simulink model "Shepherd_Battery_Model"  (R2025b)
settings: Solver=ode23  StartTime=0.0  StopTime=1000  MaxStep=0.01  RelTol=1e-4  AbsTol=1e-6
libraries: fl_lib x5, nesl_utility x5
settings Model: Creator=psvan  LastModifiedBy=psvan

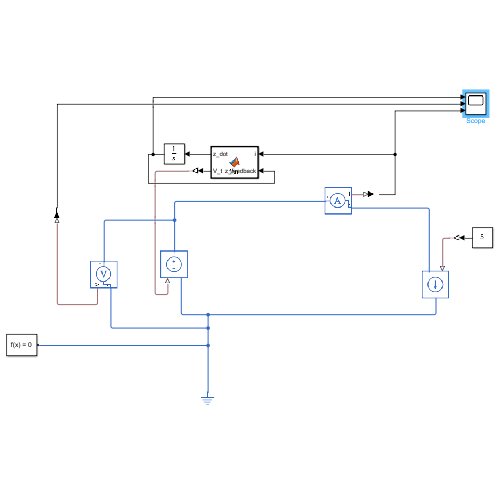
[thumbnail: Simulink's stored preview of the top-level diagram]
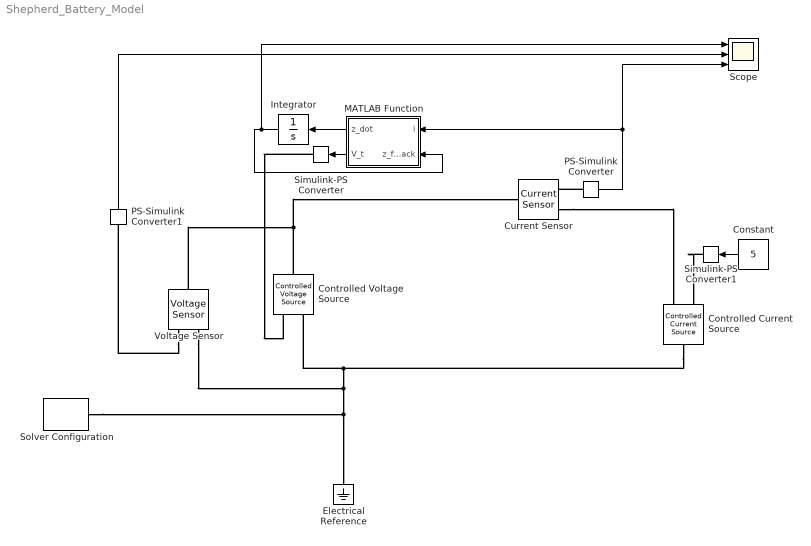
== system Shepherd_Battery_Model ==
  Constant : Constant  Value=5
  Controlled Current Source : fl_lib/Electrical/Electrical Sources/Controlled Current Source
  Controlled Voltage Source : fl_lib/Electrical/Electrical Sources/Controlled Voltage Source
  Current Sensor : fl_lib/Electrical/Electrical Sensors/Current Sensor
  Electrical Reference : fl_lib/Electrical/Electrical Elements/Electrical Reference
  Integrator : Integrator  InitialCondition=0.5
  MATLAB Function : MATLAB Function  TreatAsAtomicUnit=on
  PS-Simulink Converter : nesl_utility/PS-Simulink Converter  PhysicalDomain=network_engine_domain  SubClassName=ps_output  LeftPortType=input  RightPortType=output  PseudoPeriodic=off  Frequencies=[]  VectorFormat=inherit  Unit=inherit  AffineConversion=off
  PS-Simulink Converter1 : nesl_utility/PS-Simulink Converter  PhysicalDomain=network_engine_domain  SubClassName=ps_output  LeftPortType=input  RightPortType=output  PseudoPeriodic=off  Frequencies=[]  VectorFormat=inherit  Unit=inherit  AffineConversion=off
  Scope : Scope  NumInputPorts=3
      settings: ActiveDisplayString=3  ActiveDisplayYMinimum=4  ActiveDisplayYMaximum=6  YLabel=Current
  Simulink-PS Converter : nesl_utility/Simulink-PS Converter  PhysicalDomain=network_engine_domain  SubClassName=ps_input  LeftPortType=input  RightPortType=output  PseudoPeriodic=off  Frequencies=[]  NoiseDistribution=none  NoiseParameters=[]  Unit=1  AffineConversion=off  FilteringAndDerivatives=provide  SimscapeFilterOrder=1  InputFilterTimeConstant=0.001  UdotUserProvided=0
  Simulink-PS Converter1 : nesl_utility/Simulink-PS Converter  PhysicalDomain=network_engine_domain  SubClassName=ps_input  LeftPortType=input  RightPortType=output  PseudoPeriodic=off  Frequencies=[]  NoiseDistribution=none  NoiseParameters=[]  Unit=1  AffineConversion=off  FilteringAndDerivatives=provide  SimscapeFilterOrder=1  InputFilterTimeConstant=0.001  UdotUserProvided=0
  Solver Configuration : nesl_utility/Solver Configuration  PhysicalDomain=network_engine_domain  SubClassName=solver  LeftPortType=input  RightPortType=generic  Tones=[]  Harmonics=[]  SimulateNoise=off  Profile=off  UseLocalSampling=off  EnableSwitchedLinearOptims=on  FrequencyDomain=off  UseCCode=off  RelTol=0.001  AbsTol=0.001  MinStep=1e-09  ToWorkspace=off  RevertToSquareIcSolve=off  NumHomotopyIterations=100  PhasorMode=off  PhasorModeNumHarmonics=1  ConsistencySolver=NEWTON_XTOL_AFTER_FTOL  IndexReductionMethod=DerivativeReplacement  DoDC=off  ResidualTolerance=1e-09  ConsistencyTolSource=GLOBAL  ConsistencyAbsTol=0.001  ConsistencyRelTol=0.001  ConsistencyTolFactor=0.001  UseLocalSolver=off  LocalSolverChoice=NE_BACKWARD_EULER_ADVANCER  ResolveIndetEquations=on  FunctionEvalNumThread=1  LocalSolverSampleTime=0.001  DoFixedCost=off  MaxNonlinIter=3  MaxModeIter=2  ComputeImpulses=off  ImpulseIterations=2  LinearAlgebra=auto  LinearAlgebraNumThread=0  EquationFormulation=NE_TIME_EF  DelaysMemoryBudget=1024  AutomaticFiltering=on  FilteringTimeConstant=0.001  PartitionStorageMethod=AS_NEEDED  PartitionMemoryBudget=1024  PartitionMethod=ROBUST  MultibodyUseLocalSolver=off  MultibodyLocalSolverChoice=ODE1  MultibodyLocalSolverSampleTime=0.001
  Voltage Sensor : fl_lib/Electrical/Electrical Sensors/Voltage Sensor
  wires:
  PS-Simulink Converter1/1 -> Scope/2
  PS-Simulink Converter/1 -> Scope/3, MATLAB Function/1(i)
  Constant/1 -> Simulink-PS Converter1/1
  MATLAB Function/2(V_t) -> Simulink-PS Converter/1
  MATLAB Function/1(z_dot) -> Integrator/1
  Integrator/1 -> Scope/1, MATLAB Function/2(z_feedback)
  connections:
  Solver Configuration/RConn1 -- Voltage Sensor/RConn2 -- Controlled Voltage Source/RConn2 -- Controlled Current Source/LConn1 -- Electrical Reference/LConn1
  Controlled Voltage Source/LConn1 -- Voltage Sensor/LConn1 -- Current Sensor/LConn1
  Simulink-PS Converter/RConn1 -- Controlled Voltage Source/RConn1
  Voltage Sensor/RConn1 -- PS-Simulink Converter1/LConn1
  Current Sensor/RConn2 -- Controlled Current Source/RConn2
  PS-Simulink Converter/LConn1 -- Current Sensor/RConn1
  Simulink-PS Converter1/RConn1 -- Controlled Current Source/RConn1

== matlab function Shepherd_Battery_Model/MATLAB Function ==
  data: i input; z_dot output; z_feedback input; V_t output
function [z_dot, V_t] = fcn(i, z_feedback)

Q = 3600;      
eta = 0.995;   
E0 = 4.1;      
R_int = 0.02;  
K = 0.01;      
A = 0.1;       
B = 0.5;       

if z_feedback < 0.01
    z = 0.01;
else
    z = z_feedback;
end

z_dot = -(eta * i) / Q;
term1 = E0;
term2 = R_int * i;
term3 = K * (1/z) * i;
term4 = K * ((1 - z) / z);
term5 = A * exp(-B * Q/3600 * (1 - z)); 

V_t = term1 - term2 - term3 - term4 + term5;

end
